simulink model "extra_tip_sim"  (Simulink 9.0)
settings: Solver=FixedStepDiscrete  StartTime=start_time  StopTime=stop_time  FixedStep=0.020  RelTol=1e-3  EnableMultiTasking=on
InitFcn:
  | extra_tip_sim_init
values from neighbouring files (symbols this model uses):
  bucketAngle = WeighDebug_TOAbucket_angle_t27    [extra_tip_sim_init.m]
  imuX = WeighDebug_TOAeef_imu_accelX_t27    [extra_tip_sim_init.m]    (also in imu_pitch_cal_sim_init.m = WeighDebug_TOAeef_imu_accelX_t194)
  imuY = WeighDebug_TOAeef_imu_accelY_t27    [extra_tip_sim_init.m]    (also in imu_pitch_cal_sim_init.m = WeighDebug_TOAeef_imu_accelY_t194)
  imuZ = WeighDebug_TOAeef_imu_accelZ_t27    [extra_tip_sim_init.m]    (also in imu_pitch_cal_sim_init.m = WeighDebug_TOAeef_imu_accelZ_t194)
  liftAngle = WeighDebug_TOAlift_angle_t27    [extra_tip_sim_init.m]    (also in imu_pitch_cal_sim_init.m = WeighDebug_TOAlift_angle_t194)
  liftCmd = WeighDebug_TOAlift_valve_cmd_t27    [extra_tip_sim_init.m]
  liftCylLength = WeighDebug_LiftCylNormLen_t27    [extra_tip_sim_init.m]    (also in imu_pitch_cal_sim_init.m = WeighDebug_LiftCylLenghtNorm_Val_t194)
  liftCylPress = WeighDebug_LiftCylPres_t27    [extra_tip_sim_init.m]    (also in imu_pitch_cal_sim_init.m = WeighDebug_LiftCylPres_t194)
  payloadTarget = TOAtestPts_toa_payload_target_final_t27    [extra_tip_sim_init.m]
  steerAng = WeighDebug_TOAsteering_angle_t27    [extra_tip_sim_init.m]    (also in imu_pitch_cal_sim_init.m = WeighDebug_TOAsteering_angle_t194)
  tiltCmd = WeighDebug_TOAtilt_valve_cmd_t27    [extra_tip_sim_init.m]
  tiltExt = WeighDebug_TOAtilt_extension_t27    [extra_tip_sim_init.m]    (also in imu_pitch_cal_sim_init.m = WeighDebug_TOAtilt_extension_t194)
  tiltHePress = WeighDebug_TOAtilt_he_pressure_t27    [extra_tip_sim_init.m]    (also in imu_pitch_cal_sim_init.m = WeighDebug_TOAtilt_he_pressure_t194)
  tiltRePress = WeighDebug_TOAtilt_re_pressure_t27    [extra_tip_sim_init.m]    (also in imu_pitch_cal_sim_init.m = WeighDebug_TOAtilt_re_pressure_t194)
  time = t27    [extra_tip_sim_init.m]    (also in imu_pitch_cal_sim_init.m = t194)
  time2 = t27    [extra_tip_sim_init.m]    (also in imu_pitch_cal_sim_init.m = t194)
  time3 = t28    [extra_tip_sim_init.m]
  toolMass = WeighDebug_TOAtool_mass_t28    [extra_tip_sim_init.m]
  unlatchTrigger = WeighDebug_TOAunlatch_trigger_t27    [extra_tip_sim_init.m]
undefined symbols (not defined in the file or in its folder): g, timestep, TipAssistLiveWeighStatus_t, TipAssistPfwStatus_t, toa_appNumber, toa_imu_lpf_cutoff_hz, toa_imuBasicOrient, toa_liftBoreDia, toa_liveLpfCutoffHz, toa_pfwLpfCutoffHz, toa_ratedPayload, toa_tiltBoreDia, toa_tiltNumCyl, toa_tiltRodDia, toa_toolBcLength
libraries: simulink x28, lib_CATutils_Utilities_ApplyName_v2 x15, lib_CATutils_Filters_1Pole_LowPass x3, tip_assist_lib x3, lib_CATutils_Timer_Countdown x3, simulink_extras x2, lib_CATutils_Override x1
(part 3 of 3)

== matlab function Tip-Off Assist Payload/Pseudo-Frictionless Weigh/Statistics Estimation/MATLAB Function ==
  data: newSample input double; meanEst output double; stdevEst output double; filterFactor input double; reset input double
function [meanEst, stdevEst] = fcn(newSample, filterFactor, reset)
% Implements a running mean and standard deviation estimate.
% Formula from:
%   Estimation of Variance by a Recursive Equation
%   by M. Melvin Bruce, October 1969, Langley Research Center (NASA)
% Adapted from PCS's pcs_io.c file.

persistent lastMeanEst lastVarianceEst;

% Init to a high variance to ensure confidence is initially low.
% Note that the choice of mean initialization value determines to which
% side the weight will err.
if isempty(lastMeanEst) || reset
    lastMeanEst = single(newSample);
    lastVarianceEst = single(20);
end

A = 1 - filterFactor;   % "A" from the NASA paper
meanEst = A * lastMeanEst + (1.0 - A) * newSample;
varianceEst = A * lastVarianceEst + (1.0 - A) * (1.0 + A) * (newSample - lastMeanEst) * (newSample - lastMeanEst) / 2.0;
stdevEst = sqrt(varianceEst);

% For next time...
lastMeanEst = meanEst;
lastVarianceEst = varianceEst;
end

== matlab function Tip-Off Assist Payload/Pseudo-Frictionless Weigh/Variance Anti-Noise Filter/MATLAB Function ==
  data: u input double; y output double; reset input double
function y = movingAverage(u, reset)

persistent lastSample
if isempty(lastSample) || reset
    lastSample = single(u);
end
y = (u + lastSample) / 2;
lastSample = u;

== matlab function Tip-Off Assist Payload/Pseudo-Frictionless Weigh/Statistics Estimation1/MATLAB Function ==
  data: newSample input double; meanEst output double; stdevEst output double; filterFactor input double; reset input double; resetSample input double; resetVariance input double
function [meanEst, stdevEst] = fcn(newSample, filterFactor, reset, resetSample, resetVariance)
% Implements a running mean and standard deviation estimate.
% Formula from:
%   Estimation of Variance by a Recursive Equation
%   by M. Melvin Bruce, October 1969, Langley Research Center (NASA)
% Adapted from PCS's pcs_io.c file.

persistent lastMeanEst lastVarianceEst;

% Init to a high variance to ensure confidence is initially low.
% Init to a high mean so the true value is always approached from above,
% which will ensure a non-warmed-up filter errs high, which will cause
% Tip-Off Assist to err low to prevent truck overload.
if isempty(lastMeanEst) || reset
    lastMeanEst = single(resetSample);
    lastVarianceEst = single(resetVariance);
end

A = 1 - filterFactor;   % "A" from the NASA paper
meanEst = A * lastMeanEst + (1.0 - A) * newSample;
varianceEst = A * lastVarianceEst + (1.0 - A) * (1.0 + A) * (newSample - lastMeanEst) * (newSample - lastMeanEst) / 2.0;
stdevEst = sqrt(varianceEst);

% For next time...
lastMeanEst = meanEst;
lastVarianceEst = varianceEst;
end

== matlab function Tip-Off Assist Payload/Pseudo-Frictionless Weigh/Variance Anti-Noise Filter1/MATLAB Function ==
  data: u input double; y output double; reset input double
function y = movingAverage(u, reset)

persistent lastSample
if isempty(lastSample) || reset
    lastSample = u;
end
y = (u + lastSample) / 2;
lastSample = u;

== stateflow chart Tip-Off Assist Payload/Pseudo-Frictionless Weigh/Notch filter/NotchFilter/Filter ==
  state Update
    du: updateFilter();
  state initFilter [function]
    (default) -> (junction 133) : {
        | q = (cf*cf*ts*ts)/4.0c;
        | r = cf*ts;
        | p = 1.0c + q;
        | s = 2.0c * (q - 1.0c);
        | t = p + r;
        |
        | alpha = p / t;
        | beta = s / t;
        | gamma = r / t;
        | }
    (junction 133) -> (junction 134) : {
        | rawHist[0] = raw;
        | rawHist[1] = raw;
        | rawHist[2] = raw;
        | }
    (junction 134) -> (junction 135) : {
        | filtHist[0] = raw;
        | filtHist[1] = raw;
        | filtHist[2] = raw;
        | }
    (junction 135) -> (junction 136) : {
        | filtered = filtHist[0];
        | }
  state updateFilter [function]
    (default) -> (junction 141) : {
        | rawHist[2] = rawHist[1];
        | rawHist[1] = rawHist[0];
        | rawHist[0] = raw;
        | }
    (junction 141) -> (junction 142) : {
        | filtHist[2] = filtHist[1];
        | filtHist[1] = filtHist[0];
        | filtHist[0] = (alpha * (rawHist[0] + rawHist[2] - filtHist[2])) + (beta * (rawHist[1] - filtHist[1])) + (gamma * filtHist[2]);
        | }
    (junction 142) -> (junction 143) : {
        | filtered = filtHist[0];
        | }
  (default) -> (junction 157)
  Update -> (junction 157) : [reset]
  (junction 157) -> Update : {initFilter();}
  data: q temporary single; r temporary single; p temporary single; s temporary single; t temporary single; raw input single; reset input boolean; ts input single; cf input single; filtered output single; rawHist local single size=3; filtHist local single size=3; alpha local single; beta local single; gamma local single

== stateflow chart Tip-Off Assist Payload/Pseudo-Frictionless Weigh/Notch filter/NotchFilter1/Filter ==
  state Update
    du: updateFilter();
  state initFilter [function]
    (default) -> (junction 171) : {
        | q = (cf*cf*ts*ts)/4.0c;
        | r = cf*ts;
        | p = 1.0c + q;
        | s = 2.0c * (q - 1.0c);
        | t = p + r;
        |
        | alpha = p / t;
        | beta = s / t;
        | gamma = r / t;
        | }
    (junction 171) -> (junction 172) : {
        | rawHist[0] = raw;
        | rawHist[1] = raw;
        | rawHist[2] = raw;
        | }
    (junction 172) -> (junction 173) : {
        | filtHist[0] = raw;
        | filtHist[1] = raw;
        | filtHist[2] = raw;
        | }
    (junction 173) -> (junction 174) : {
        | filtered = filtHist[0];
        | }
  state updateFilter [function]
    (default) -> (junction 179) : {
        | rawHist[2] = rawHist[1];
        | rawHist[1] = rawHist[0];
        | rawHist[0] = raw;
        | }
    (junction 179) -> (junction 180) : {
        | filtHist[2] = filtHist[1];
        | filtHist[1] = filtHist[0];
        | filtHist[0] = (alpha * (rawHist[0] + rawHist[2] - filtHist[2])) + (beta * (rawHist[1] - filtHist[1])) + (gamma * filtHist[2]);
        | }
    (junction 180) -> (junction 181) : {
        | filtered = filtHist[0];
        | }
  (default) -> (junction 195)
  Update -> (junction 195) : [reset]
  (junction 195) -> Update : {initFilter();}
  data: q temporary single; r temporary single; p temporary single; s temporary single; t temporary single; raw input single; reset input boolean; ts input single; cf input single; filtered output single; rawHist local single size=3; filtHist local single size=3; alpha local single; beta local single; gamma local single

== stateflow chart Tip-Off Assist Payload/Pseudo-Frictionless Weigh/Notch filter/NotchFilter2/Filter ==
  state Update
    du: updateFilter();
  state initFilter [function]
    (default) -> (junction 209) : {
        | q = (cf*cf*ts*ts)/4.0c;
        | r = cf*ts;
        | p = 1.0c + q;
        | s = 2.0c * (q - 1.0c);
        | t = p + r;
        |
        | alpha = p / t;
        | beta = s / t;
        | gamma = r / t;
        | }
    (junction 209) -> (junction 210) : {
        | rawHist[0] = raw;
        | rawHist[1] = raw;
        | rawHist[2] = raw;
        | }
    (junction 210) -> (junction 211) : {
        | filtHist[0] = raw;
        | filtHist[1] = raw;
        | filtHist[2] = raw;
        | }
    (junction 211) -> (junction 212) : {
        | filtered = filtHist[0];
        | }
  state updateFilter [function]
    (default) -> (junction 217) : {
        | rawHist[2] = rawHist[1];
        | rawHist[1] = rawHist[0];
        | rawHist[0] = raw;
        | }
    (junction 217) -> (junction 218) : {
        | filtHist[2] = filtHist[1];
        | filtHist[1] = filtHist[0];
        | filtHist[0] = (alpha * (rawHist[0] + rawHist[2] - filtHist[2])) + (beta * (rawHist[1] - filtHist[1])) + (gamma * filtHist[2]);
        | }
    (junction 218) -> (junction 219) : {
        | filtered = filtHist[0];
        | }
  (default) -> (junction 233)
  Update -> (junction 233) : [reset]
  (junction 233) -> Update : {initFilter();}
  data: q temporary single; r temporary single; p temporary single; s temporary single; t temporary single; raw input single; reset input boolean; ts input single; cf input single; filtered output single; rawHist local single size=3; filtHist local single size=3; alpha local single; beta local single; gamma local single

== matlab function Tip-Off Assist Payload/Pseudo-Frictionless Weigh/Statistics Estimation1/Two Sided St. Dev. from Bound ==
  data: confidence input double; stdev output double; bound input double
function stdev = TwoSidedConfBound(confidence, bound)
% Calculates the st. dev. of a confidence interval in terms of half its width.
%
% Inputs:
%   confidence
%   Confidence that the input bound will enclose the true value.
%
%   bound
%   Bound of the confidence interval, expressed in the same units as stdev.
%   
%   For lower bound, the true value will lie above the mean minus this
%   value.
%   The opposite is true for an upper bound.
%
%   Potential units for the arguments are percent of rated payload or
%   payload.
%
% Outputs:
%   stdev
%   The standard deviation, expressed in the same units as
%   bound, that corresponds to the given bound. Can be thought of as
%   describing the scale of the normal distribution whose confidence
%   interval with given bounds results in the given confidence.
%   
% Inspired from pcs_calculate_confidence() in pcs_io.c

% Table of confidence vs two-sided confidence interval bound.
% Units of confidence decimal percent and the ratio of standard
% deviation of a standard normal distribution.
xConfidenceTwoSided = [ 0.0, 0.235822844, 0.382924922, 0.516072694, 0.631879747, 0.728667676, 0.806398927, 0.866385543, 0.910869057, 0.942566872, 0.964271153, 0.978551778, 0.987580668, 0.993066052, 0.997300204, 0.999534742, 1.0 ];
yStdevRatio = [ 0.0, 0.3, 0.5, 0.7, 0.9, 1.1, 1.3, 1.5, 1.7, 1.9, 2.1, 2.3, 2.5, 2.7, 3.0, 3.5, 4.0 ];
stdev_ratio = interp1(xConfidenceTwoSided, yStdevRatio, confidence);
stdev = bound / stdev_ratio;
